simulink subsystem "KeplerianOrbit"  (R2024b)
settings: Solver=VariableStepAuto  StartTime=0.0  StopTime=10.0  RelTol=1e-3
settings Model: Creator=marco  LastModifiedBy=ferru

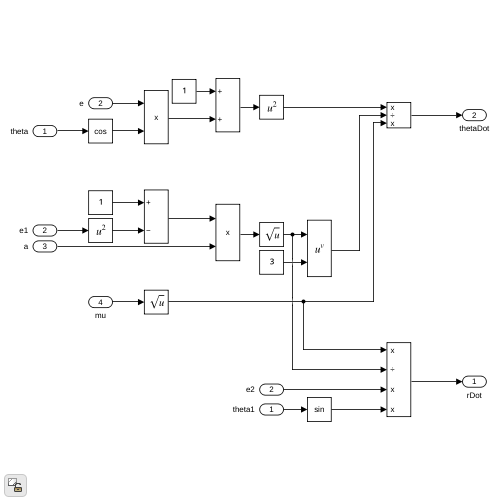
[thumbnail: Simulink's stored preview of the top-level diagram]
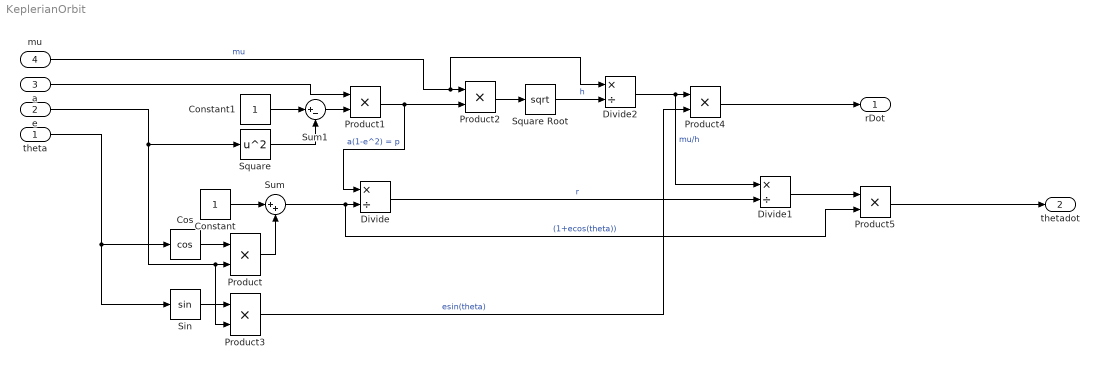
== system KeplerianOrbit ==
  theta : Inport
  e : Inport  Port=2
  a : Inport  Port=3
  mu : Inport  Port=4
  Constant : Constant
  Constant1 : Constant
  Cos : Trigonometry  Operator=cos
  Divide : Product  Inputs=*/
  Divide1 : Product  Inputs=*/
  Divide2 : Product  Inputs=*/
  Product{,1..5} (6 alike) : Product
  Sin : Trigonometry
  Square : Math  Operator=square
  Square Root : Sqrt
  Sum : Sum  Inputs=|++
  Sum1 : Sum  Inputs=|+-
  rDot : Outport
  thetadot : Outport  Port=2
  wires:
  Constant/1 -> Sum/1
  theta/1 -> Sin/1, Cos/1
  Cos/1 -> Product/1
  e/1 -> Product/2, Product3/2, Square/1
  Product/1 -> Sum/2
  Sum/1 -> Divide/2, Product5/2  "(1+ecos(theta))"
  Constant1/1 -> Sum1/1
  Square/1 -> Sum1/2
  Sum1/1 -> Product1/2
  a/1 -> Product1/1
  Product1/1 -> Divide/1, Product2/2  "a(1-e^2) = p"
  Divide/1 -> Divide1/2  "r"
  mu/1 -> Product2/1, Divide2/1  "mu"
  Product2/1 -> Square Root/1
  Square Root/1 -> Divide2/2  "h"
  Sin/1 -> Product3/1
  Divide2/1 -> Product4/1, Divide1/1  "mu/h"
  Product3/1 -> Product4/2  "esin(theta)"
  Product4/1 -> rDot/1
  Divide1/1 -> Product5/1
  Product5/1 -> thetadot/1
